simulink model "Sistema_completo_original"  (R2026a)
settings: Solver=FixedStepAuto  StopTime=Tsim  FixedStep=Ts
InitFcn:
  | sys_params
values from neighbouring files (symbols this model uses):
  D = 20    [sys_params.m]    (also in sys_params_original.m)
  fLO = fc_rx + fIF    (= 2340000)    [sys_params.m]    (also in sys_params_original.m)
  fsub = P('fsub')    [radio_gui.m]    (also in radio_guiV2.m; sys_params.m = [fc1 fc2 fc3]; sys_params_original.m = [20e3 60e3 100e3])
  K_FDM = 1/3    (= 0.333333333333)    [sys_params.m]    (also in sys_params_original.m)
  phi = -2*pi*fsub*tau    [calibrate.m]    (also in phi.mat = [-6.55022068273 -7.86026481928 -10.0436717135]; sys_params.m = zeros(1,3); sys_params_original.m = zeros(1,3))
  Ts = 1/Fs    (= 5e-08)    [sys_params.m]    (also in sys_params_original.m = 2e-06)
  Ts2 = 1/Fs2    (= 1e-06)    [sys_params.m]    (also in sys_params_original.m = 4e-05)
undefined symbols (not defined in the file or in its folder): designMultirateFIR
libraries: commanapbnd3 x5, dsparch4 x3, dspfdesign x2, dspmlti4 x2
settings Model: Creator=felipe  LastModifiedBy=felipe

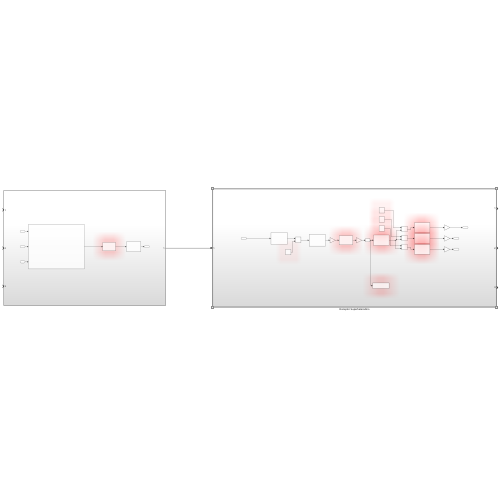
[thumbnail: Simulink's stored preview of the top-level diagram]
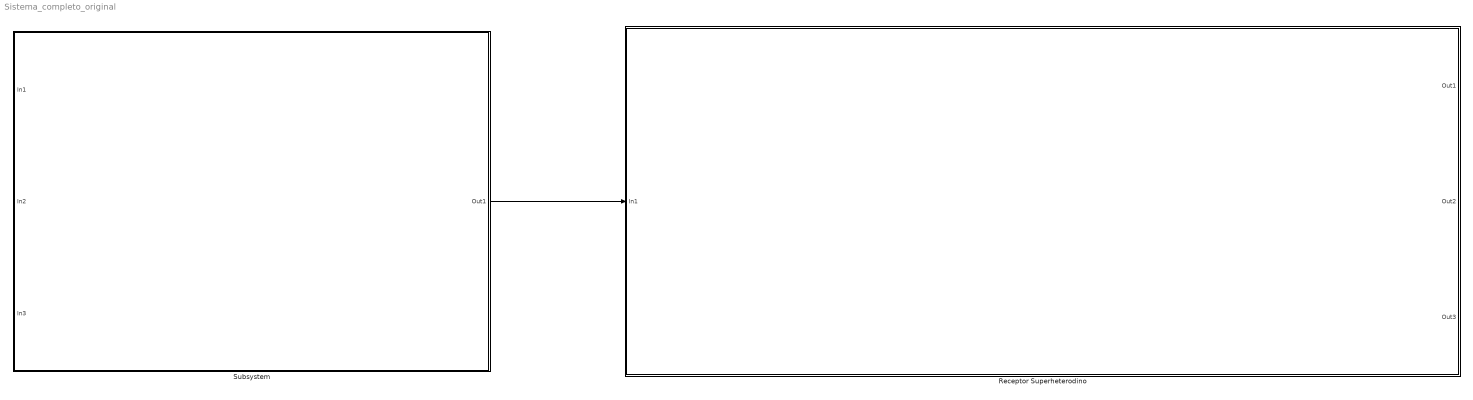
== system Sistema_completo_original ==
  Receptor Superheterodino : Subsystem
  Subsystem : Subsystem
  wires:
  Subsystem/1(Out1) -> Receptor Superheterodino/1(In1)

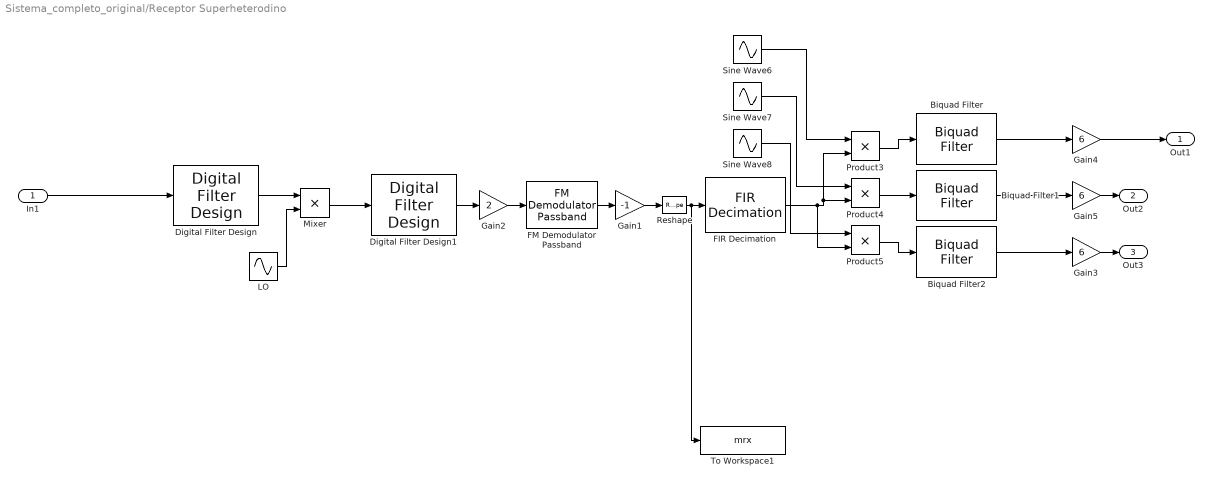
== system Sistema_completo_original/Receptor Superheterodino ==
  In1 : Inport
  Biquad Filter : dsparch4/Biquad Filter  FilterSource=Dialog parameters  CoeffSource=Specify via dialog  FilterObject=BQF  IIRFiltStruct=Direct form II transposed  BiQuadCoeffs=sosAud  ScaleValues=1  IC=0  ICnum=0  ICden=0  a0Flag=Warning  optimizeScaleValues=on  ScaleValueMode=Specify via input port (g)  InputProcessing=Columns as channels (frame based)  roundingMode=Floor  overflowMode=off  scaleValueFracLength=14  denProdOutputFracLength=30  denAccumFracLength=30  secondMemoryFracLength=15
  Biquad Filter1 : dsparch4/Biquad Filter  FilterSource=Dialog parameters  CoeffSource=Specify via dialog  FilterObject=BQF  IIRFiltStruct=Direct form II transposed  BiQuadCoeffs=sosAud  ScaleValues=1  IC=0  ICnum=0  ICden=0  a0Flag=Warning  optimizeScaleValues=on  ScaleValueMode=Specify via input port (g)  InputProcessing=Columns as channels (frame based)  roundingMode=Floor  overflowMode=off  scaleValueFracLength=14  denProdOutputFracLength=30  denAccumFracLength=30  secondMemoryFracLength=15
  Biquad Filter2 : dsparch4/Biquad Filter  FilterSource=Dialog parameters  CoeffSource=Specify via dialog  FilterObject=BQF  IIRFiltStruct=Direct form II transposed  BiQuadCoeffs=sosAud  ScaleValues=1  IC=0  ICnum=0  ICden=0  a0Flag=Warning  optimizeScaleValues=on  ScaleValueMode=Specify via input port (g)  InputProcessing=Columns as channels (frame based)  roundingMode=Floor  overflowMode=off  scaleValueFracLength=14  denProdOutputFracLength=30  denAccumFracLength=30  secondMemoryFracLength=15
  Digital Filter Design : dspfdesign/Digital Filter Design  mwdsp_browser_bugfix_var=off
  Digital Filter Design1 : dspfdesign/Digital Filter Design  mwdsp_browser_bugfix_var=off
  FIR Decimation : dspmlti4/FIR Decimation  FilterSource=Dialog parameters  h=hDec  D=D  filtStruct=Direct form  FilterObject=FDECIM  framing=Enforce single-rate processing  AllowArbitraryInputLength=off  inputOffset=0  outputBufInitCond=0  roundingMode=Floor  overflowMode=off  firstCoeffDataTypeStr=Inherit: Same word length as input  firstCoeffMin=[]  firstCoeffMax=[]  firstCoeffLastDataTypeStr=Inherit: Same word length as input  outputDataTypeStr=Inherit: Same as accumulator  outputMin=[]  outputMax=[]  outputLastDataTypeStr=Inherit: Same as accumulator
  FM Demodulator Passband : commanapbnd3/FM Demodulator Passband  Fc=fIF  Ph=0  Kc=df  Ho=1000
  Gain1 : Gain  Gain=-1
  Gain2 : Gain  Gain=2
  Gain3 : Gain  Gain=6
  Gain4 : Gain  Gain=6
  Gain5 : Gain  Gain=6
  LO : Sin  Frequency=2*pi*fLO  SampleTime=Ts
  Mixer : Product
  Product3 : Product
  Product4 : Product
  Product5 : Product
  Reshape : Reshape
  Sine Wave6 : Sin  Frequency=2*pi*fsub(1)  Phase=phi(1)  SampleTime=Ts2
  Sine Wave7 : Sin  Frequency=2*pi*fsub(2)  Phase=phi(2)  SampleTime=Ts2
  Sine Wave8 : Sin  Frequency=2*pi*fsub(3)  Phase=phi(3)  SampleTime=Ts2
  To Workspace1 : ToWorkspace  VariableName=mrx  SampleTime=Ts
  Out1 : Outport
  Out2 : Outport  Port=2
  Out3 : Outport  Port=3
  wires:
  Gain3/1 -> Out3/1
  FM Demodulator Passband/1 -> Gain1/1
  Mixer/1 -> Digital Filter Design1/1
  Digital Filter Design/1 -> Mixer/1
  Gain4/1 -> Out1/1
  In1/1 -> Digital Filter Design/1
  Reshape/1 -> To Workspace1/1, FIR Decimation/1
  Sine Wave6/1 -> Product3/1
  Product3/1 -> Biquad Filter/1
  Gain2/1 -> FM Demodulator Passband/1
  Digital Filter Design1/1 -> Gain2/1
  Biquad Filter1/1 -> Gain5/1
  Biquad Filter2/1 -> Gain3/1
  Product4/1 -> Biquad Filter1/1
  Sine Wave8/1 -> Product5/1
  Product5/1 -> Biquad Filter2/1
  Biquad Filter/1 -> Gain4/1
  FIR Decimation/1 -> Product4/2, Product3/2, Product5/2
  LO/1 -> Mixer/2
  Gain5/1 -> Out2/1
  Sine Wave7/1 -> Product4/1
  Gain1/1 -> Reshape/1

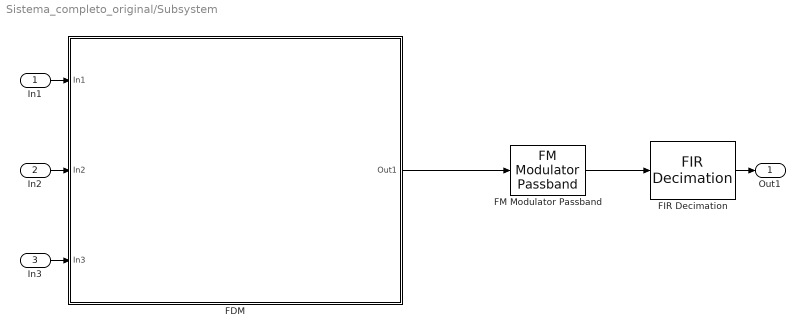
== system Sistema_completo_original/Subsystem ==
  In1 : Inport
  In2 : Inport  Port=2
  In3 : Inport  Port=3
  FDM : Subsystem
  FIR Decimation : dspmlti4/FIR Decimation  FilterSource=Auto  h=designMultirateFIR(1,2)  D=20  filtStruct=Direct form  FilterObject=FDECIM  framing=Allow multirate processing  AllowArbitraryInputLength=off  inputOffset=0  outputBufInitCond=0  roundingMode=Floor  overflowMode=off  firstCoeffDataTypeStr=Inherit: Same word length as input  firstCoeffMin=[]  firstCoeffMax=[]  firstCoeffLastDataTypeStr=Inherit: Same word length as input  outputDataTypeStr=Inherit: Same as accumulator  outputMin=[]  outputMax=[]  outputLastDataTypeStr=Inherit: Same as accumulator
      settings: LibrarySourceBlock=|
      | dsphdlsupportfiltering/FIR
      | Decimation
  FM Modulator Passband : commanapbnd3/FM Modulator Passband  Fc=fc_tx  Ph=0  Kc=deltaf
  Out1 : Outport
  wires:
  FDM/1(Out1) -> FM Modulator Passband/1
  In2/1 -> FDM/2(In2)
  FIR Decimation/1 -> Out1/1
  In3/1 -> FDM/3(In3)
  FM Modulator Passband/1 -> FIR Decimation/1
  In1/1 -> FDM/1(In1)

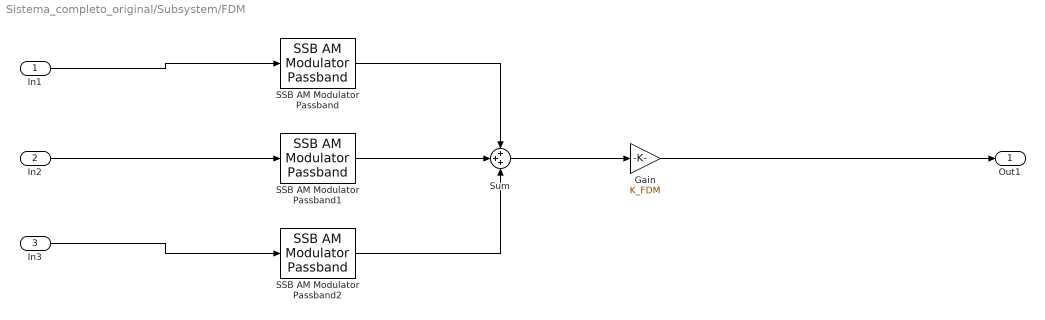
== system Sistema_completo_original/Subsystem/FDM ==
  In1 : Inport
  In2 : Inport  Port=2
  In3 : Inport  Port=3
  Gain : Gain  Gain=K_FDM
  SSB AM Modulator Passband : commanapbnd3/SSB AM Modulator Passband  Fc=fc1  Ph=0  Sd=Upper  Ho=Nh
  SSB AM Modulator Passband1 : commanapbnd3/SSB AM Modulator Passband  Fc=fc2  Ph=0  Sd=Upper  Ho=Nh
  SSB AM Modulator Passband2 : commanapbnd3/SSB AM Modulator Passband  Fc=fc3  Ph=0  Sd=Upper  Ho=Nh
  Sum : Sum  Inputs=+++
  Out1 : Outport
  wires:
  SSB AM Modulator Passband1/1 -> Sum/2
  SSB AM Modulator Passband2/1 -> Sum/3
  Sum/1 -> Gain/1
  SSB AM Modulator Passband/1 -> Sum/1
  Gain/1 -> Out1/1
  In3/1 -> SSB AM Modulator Passband2/1
  In2/1 -> SSB AM Modulator Passband1/1
  In1/1 -> SSB AM Modulator Passband/1
